simulink model "W04_J_both"  (R2024b)
settings: Solver=ode4  StartTime=0  StopTime=T_both  FixedStep=h  RelTol=1e-3
StopFcn:
  | W04_J_plot;
values from neighbouring files (symbols this model uses):
  beta_c = 0    [W04_0_setup.m]
  k_neg = cfg.k_neg    [W04_0_setup.m]
  k_pos = cfg.k_pos    [W04_0_setup.m]
  Kb_u = 1    [W04_0_setup.m]
  Kd = 100    [W04_0_setup.m]
  Ki_u = 200    [W04_0_setup.m]
  Kp = 300    [W04_0_setup.m]
  Kp_u = 200    [W04_0_setup.m]
  mp = 25    [W04_0_setup.m]
  n_max = cfg.n_max    [W04_0_setup.m]
  n_min = cfg.n_min    [W04_0_setup.m]
  N_speed = min(2*y_pont*(T_hi - X_max/2), 2*y_pont*(X_max/2 - T_lo))    [W04_0_setup.m]
  rp = [0.05 0 -0.35]'    [W04_0_setup.m]
  V_c = 0    [W04_0_setup.m]
  x0 = zeros(12,1)    [W04_0_setup.m]
  X_max = 120    [W04_0_setup.m]
  y_pont = cfg.y_pont    [W04_0_setup.m]
libraries: simulink x2
settings Model: Creator=admin  LastModifiedBy=admin
settings DataIOCC: ReturnWorkspaceOutputs=off

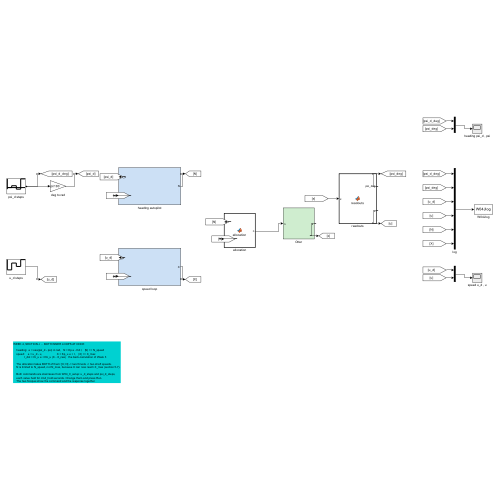
[thumbnail: Simulink's stored preview of the top-level diagram]
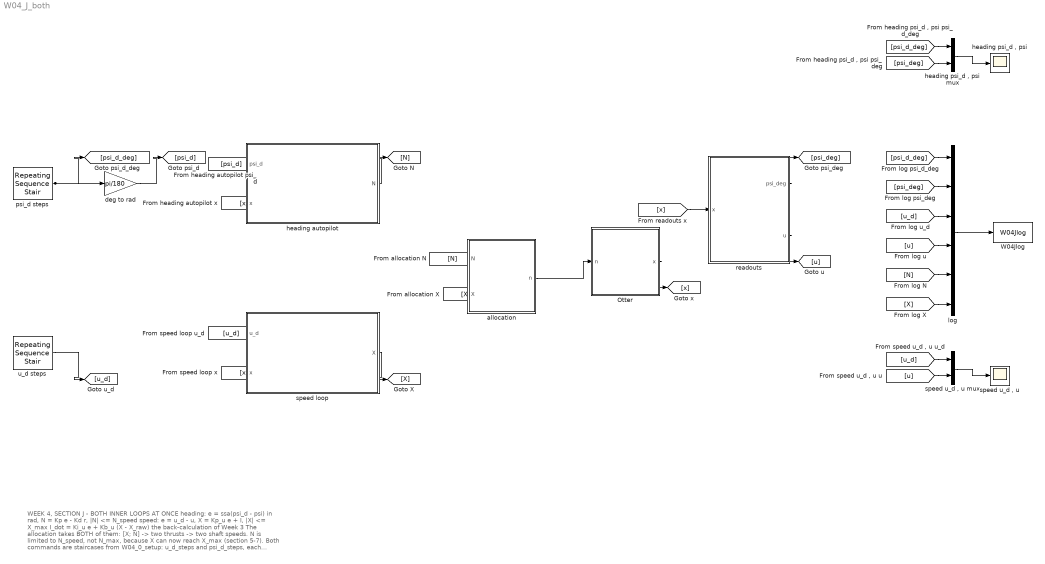
== system W04_J_both ==
  note: WEEK 4, SECTION J  -  BOTH INNER LOOPS AT ONCE
      |
      |     heading:  e = ssa(psi_d - psi) in rad,   N = Kp e - Kd r,   |N| <= N_speed
      |     speed:    e = u_d - u,                   X = Kp_u e + I,    |X| <= X_max
      |               I_dot = Ki_u e + Kb_u (X - X_raw)   the back-calculation of Week 3
      |
      |     The allocation takes BOTH of them: [X; N] -> two thrusts -> two shaft speeds.
      |     N is limited to N_speed, not N_max, because X can now reach X_max (section 5-7).
      |
      |     Both commands are staircases from W04_0_setup: u_d_steps and psi_d_steps,
      |     each value held for cmd_hold seconds. Change them and press Run.
      |     The two Scopes show the command and the response together.
  Otter : Subsystem
  W04Jlog : ToWorkspace  VariableName=W04Jlog  SaveFormat=Structure With Time  SampleTime=-1
  allocation : MATLAB Function  TreatAsAtomicUnit=on
  deg to rad : Gain  Gain=pi/180
  heading autopilot : Subsystem
  "heading psi_d , psi" : Scope
  "heading psi_d , psi mux" : Mux  Inputs=2
  log : Mux  Inputs=6
  psi_d steps : simulink/Sources/Repeating Sequence Stair  OutValues=psi_d_steps  tsamp=cmd_hold  OutMin=[]  OutMax=[]  OutDataTypeStr=double  OutputDataTypeScalingMode=double  OutDataType=fixdt(0,8)  ConRadixGroup=Best Precision: Vector-wise  OutScaling=2^-12
  readouts : MATLAB Function  TreatAsAtomicUnit=on
  speed loop : Subsystem
  "speed u_d , u" : Scope
  "speed u_d , u mux" : Mux  Inputs=2
  u_d steps : simulink/Sources/Repeating Sequence Stair  OutValues=u_d_steps  tsamp=cmd_hold  OutMin=[]  OutMax=[]  OutDataTypeStr=double  OutputDataTypeScalingMode=double  OutDataType=fixdt(0,8)  ConRadixGroup=Best Precision: Vector-wise  OutScaling=2^-12
  wires:
  psi_d steps/1 -> deg to rad/1, [psi_d_deg]
  deg to rad/1 -> [psi_d]
  u_d steps/1 -> [u_d]
  [psi_d] -> heading autopilot/1(psi_d)
  [x] -> heading autopilot/2(x)
  [u_d] -> speed loop/1(u_d)
  [x] -> speed loop/2(x)
  heading autopilot/1(N) -> [N]
  speed loop/1(X) -> [X]
  [N] -> allocation/1(N)
  [X] -> allocation/2(X)
  allocation/1(n) -> Otter/1(n)
  Otter/1(x) -> [x]
  [x] -> readouts/1(x)
  readouts/1(psi_deg) -> [psi_deg]
  readouts/2(u) -> [u]
  [psi_d_deg] -> log/1
  [psi_deg] -> log/2
  [u_d] -> log/3
  [u] -> log/4
  [N] -> log/5
  [X] -> log/6
  log/1 -> W04Jlog/1
  [psi_d_deg] -> "heading psi_d , psi mux"/1
  [psi_deg] -> "heading psi_d , psi mux"/2
  "heading psi_d , psi mux"/1 -> "heading psi_d , psi"/1
  [u_d] -> "speed u_d , u mux"/1
  [u] -> "speed u_d , u mux"/2
  "speed u_d , u mux"/1 -> "speed u_d , u"/1

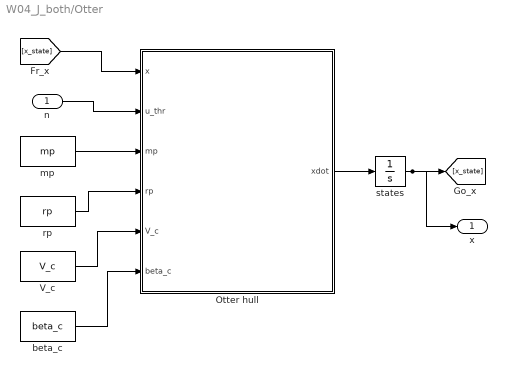
== system W04_J_both/Otter ==
  n : Inport
  Otter hull : MATLAB Function  TreatAsAtomicUnit=on
  V_c : Constant  Value=V_c
  beta_c : Constant  Value=beta_c
  mp : Constant  Value=mp
  rp : Constant  Value=rp
  states : Integrator  InitialCondition=x0
  x : Outport
  wires:
  Otter hull/1(xdot) -> states/1
  mp/1 -> Otter hull/3(mp)
  [x_state] -> Otter hull/1(x)
  beta_c/1 -> Otter hull/6(beta_c)
  n/1 -> Otter hull/2(u_thr)
  rp/1 -> Otter hull/4(rp)
  states/1 -> [x_state], x/1
  V_c/1 -> Otter hull/5(V_c)

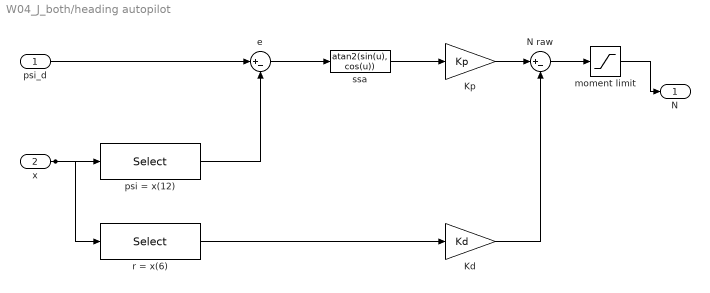
== system W04_J_both/heading autopilot ==
  psi_d : Inport
  x : Inport  Port=2
  Kd : Gain  Gain=Kd
  Kp : Gain  Gain=Kp
  N raw : Sum  Inputs=|+-
  e : Sum  Inputs=|+-
  moment limit : Saturate  UpperLimit=N_speed  LowerLimit=-N_speed
  psi = x(12) : Selector  InputPortWidth=12  IndexOptions=Index vector (dialog)  Indices=12  OutputSizes=1
  r = x(6) : Selector  InputPortWidth=12  IndexOptions=Index vector (dialog)  Indices=6  OutputSizes=1
  ssa : Fcn  Expr=atan2(sin(u), cos(u))
  N : Outport
  wires:
  x/1 -> psi = x(12)/1, r = x(6)/1
  psi_d/1 -> e/1
  psi = x(12)/1 -> e/2
  e/1 -> ssa/1
  ssa/1 -> Kp/1
  r = x(6)/1 -> Kd/1
  Kp/1 -> N raw/1
  Kd/1 -> N raw/2
  N raw/1 -> moment limit/1
  moment limit/1 -> N/1

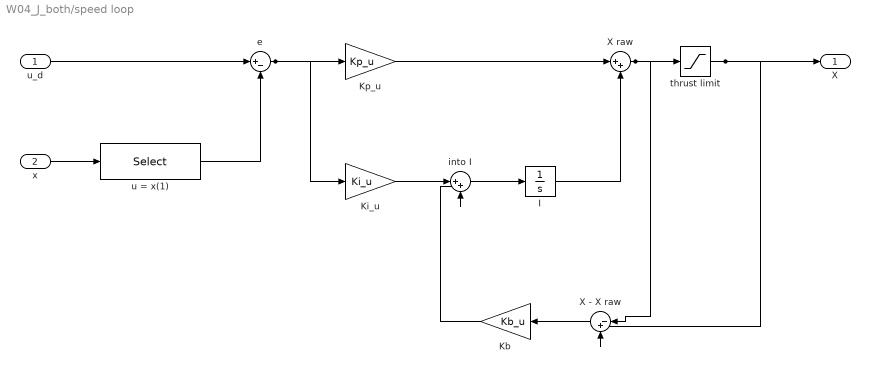
== system W04_J_both/speed loop ==
  u_d : Inport
  x : Inport  Port=2
  I : Integrator
  Kb : Gain  Gain=Kb_u
  Ki_u : Gain  Gain=Ki_u
  Kp_u : Gain  Gain=Kp_u
  X - X raw : Sum  Inputs=|-+
  X raw : Sum  Inputs=|++
  e : Sum  Inputs=|+-
  into I : Sum  Inputs=|++
  thrust limit : Saturate  UpperLimit=X_max  LowerLimit=-X_max
  u = x(1) : Selector  InputPortWidth=12  IndexOptions=Index vector (dialog)  Indices=1  OutputSizes=1
  X : Outport
  wires:
  x/1 -> u = x(1)/1
  u_d/1 -> e/1
  u = x(1)/1 -> e/2
  e/1 -> Kp_u/1, Ki_u/1
  Ki_u/1 -> into I/1
  into I/1 -> I/1
  Kp_u/1 -> X raw/1
  I/1 -> X raw/2
  X raw/1 -> thrust limit/1, X - X raw/1
  thrust limit/1 -> X/1, X - X raw/2
  X - X raw/1 -> Kb/1
  Kb/1 -> into I/2

== matlab function W04_J_both/Otter/Otter hull ==
  data: x input; xdot output double size=[12 1]; u_thr input; mp input; rp input; V_c input; beta_c input
function xdot = otter_hull(x, u_thr, mp, rp, V_c, beta_c)
% Fossen's otter.m, called unchanged from Tools/MSS/VESSELS.
%
%   x       12 states, fed back from the integrator
%   u_thr   propeller shaft speeds [rad/s]
%
% otter.m is not written for code generation, so the call is extrinsic and
% xdot has to be pre-sized for Simulink to know the output width.
coder.extrinsic('otter');

xdot = zeros(12,1);
xdot = otter(x, u_thr, mp, rp, V_c, beta_c);
end

== matlab function W04_J_both/allocation ==
  data: N input; n output double size=[2 1]; X input; y_pont parameter; k_pos parameter; k_neg parameter; n_max parameter; n_min parameter
function n = allocation(N, X, y_pont, k_pos, k_neg, n_max, n_min)
%#codegen
%ALLOCATION  전진력 X 와 요 모멘트 N 을 두 축의 회전수 n = [n_L; n_R] 로.
%            The surge force X and the yaw moment N to the two shaft speeds.
%  **두 입력 모두 제어기의 출력이다**: N 은 선수각 루프, X 는 속도 루프.
%  Both inputs are outputs of controllers: N from the heading loop, X from the
%  speed loop. In the other Week 4 models X was a constant.

% 1) 두 힘을 두 추력으로. 배치행렬 B 를 세우고 **풀면** 된다.
%    Solve B T = [X; N] rather than writing the two expressions out.
B = [1        1;              % 전진력  X = T_L + T_R        / surge force
     y_pont  -y_pont];        % 요 모멘트 N = y_pont(T_L-T_R) / yaw moment
T = B \ [X; N];               % 좌현, 우현 / port, starboard

% 2) 프로펠러 곡선 T = k n|n| 을 n 에 대해 푼다 (앞 k_pos, 뒤 k_neg).
%    Solve the propeller curve T = k n|n| for n (k_pos ahead, k_neg astern).
n = zeros(2,1);
for i = 1:2
    if T(i) >= 0
        n(i) =  sqrt( T(i) / k_pos);
    else
        n(i) = -sqrt(-T(i) / k_neg);
    end
end

% 3) 프로펠러가 낼 수 있는 범위로 자른다 (otter.m 167-170 행이 안에서 이미 자른다).
%    Clamp to what the propellers can do; otter.m clamps internally too.
n(1) = min(max(n(1), n_min), n_max);
n(2) = min(max(n(2), n_min), n_max);
end

== matlab function W04_J_both/readouts ==
  data: x input; psi_deg output double size=[1 1]; u output
function [psi_deg, u] = readouts(x)
%#codegen
%READOUTS  로그와 Scope 가 쓰는 두 값 / the two values the log and the Scopes use.
%
%  선수각은 **도** 로, 그리고 (-180, 180] 로 감아서 낸다. 감지 않으면 선회가
%  누적되어 360, 720 처럼 커지고, 명령과 겹쳐 그릴 수 없다.
%  The heading is given in degrees and wrapped into (-180, 180]; unwrapped it
%  would accumulate past 360 and could not be drawn against its command.
psi_deg = atan2(sin(x(12)), cos(x(12))) * 180/pi;
u       = x(1);
end
